simulink model "HRTF_IIR_Baris_FixedPoint_v2"  (R2025a)
settings: Solver=FixedStepDiscrete  StartTime=0.0  StopTime=T_sim  FixedStep=1/48000  RelTol=1e-3
values from neighbouring files (symbols this model uses):
  Alpha = [1 1 0.967796790113 -0.19525471365 0.941178659583 1.27759475775 0.157427422536 -0.232086624749 0.0400536246511 0.488732720219 -0.15013114138 -0.0870474720577 ... (18 elements, 2x9)]    [koeff_parameter_iir.mat]
  Beta = [1 1 4.50665299478 2.25254932437 11.1795102702 3.85997518129 18.0238230447 4.78060301042 20.7495830674 4.97041442912 17.1226318925 4.54493537547 ... (18 elements, 2x9)]    [koeff_parameter_iir.mat]
  Delay = [8966.24819844 7620.20448403]    [koeff_parameter_iir.mat]
  Gain = [4.7297619183 7.71004347236]    [koeff_parameter_iir.mat]
undefined symbols (not defined in the file or in its folder): ALPHA, BETA, DELAY, dspblkCoreblockFVToolHelper, GAIN, gcbh
settings Model: Creator=kucuk  LastModifiedBy=eoencue1
settings OptimizationCC: DefaultParameterBehavior=Inlined  EnhancedBackFolding=on  PassReuseOutputArgsAs=Individual arguments  OptimizeBlockOrder=speed  DifferentSizesBufferReuse=on  OptimizationCustomize=off  EfficientTunableParamExpr=on
settings DebuggingCC: SignalRangeChecking=warning  ParameterTunabilityLossMsg=error
settings HardwareCC: ProdBitPerPointer=32.0  ProdBitPerSizeT=32.0  ProdBitPerPtrDiffT=32.0  ProdLargestAtomicFloat=None  ProdWordSize=32.0  ProdLongLongMode=on  ProdHWDeviceType=Custom Processor->Custom
settings ModelReferenceCC: ModelReferenceNumInstancesAllowed=Single
settings SFSimCC: MATLABDynamicMemAlloc=off
settings RTWCC: SystemTargetFile=ert.tlc  GenCodeOnly=on  TemplateMakefile=ert_default_tmf  Description=Embedded Coder
settings CodeAppCC: ForceParamTrailComments=on  IgnoreCustomStorageClasses=off  OperatorAnnotations=on  SimulinkDataObjDesc=on  SFDataObjDesc=on  InsertBlockDesc=on
settings ERTTargetCC: ExtModeTransport=0.0  ExtModeStaticAlloc=off  ExtModeMexFile=ext_comm  ExtModeIntrfLevel=Level1  ERTCustomFileTemplate=example_file_process.tlc  TargetLangStandard=C99 (ISO)  SubcomponentCodeInterfacePackaging=Nonreusable function  SupportNonFinite=off

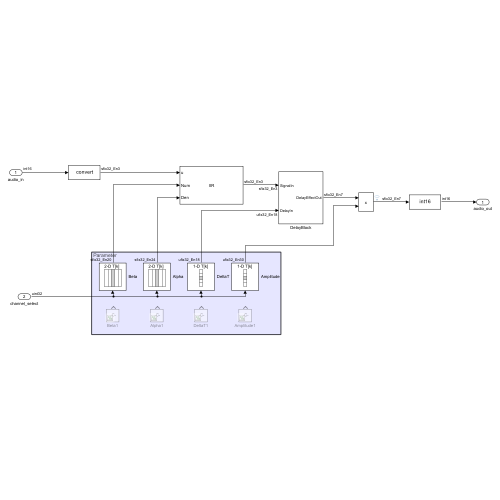
[thumbnail: Simulink's stored preview of the top-level diagram]
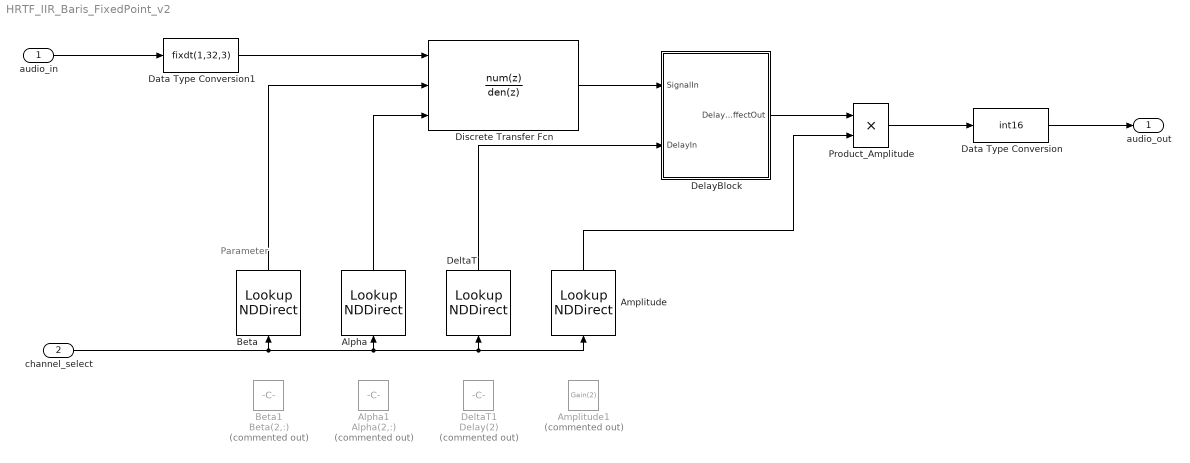
== system HRTF_IIR_Baris_FixedPoint_v2 ==
  note: Parameter
  audio_in : Inport  OutDataTypeStr=int16
  channel_select : Inport  Port=2  OutDataTypeStr=uint32
  Alpha : LookupNDDirect  InputsSelectThisObjectFromTable=Vector  Table=ALPHA  TableDataTypeStr=fixdt(1,32,24)
  Alpha1 : Constant  Commented=on  Value=Alpha(2,:)
  Amplitude : LookupNDDirect  NumberOfTableDimensions=1  Table=GAIN  TableDataTypeStr=fixdt(0,32,30)
  Amplitude1 : Constant  Commented=on  Value=Gain(2)
  Beta : LookupNDDirect  InputsSelectThisObjectFromTable=Vector  Table=BETA  TableDataTypeStr=fixdt(1,32,20)
  Beta1 : Constant  Commented=on  Value=Beta(2,:)
  Data Type Conversion : DataTypeConversion  OutDataTypeStr=int16  RndMeth=Floor
  Data Type Conversion1 : DataTypeConversion  OutDataTypeStr=fixdt(1,32,3)  RndMeth=Floor
  DelayBlock : Subsystem
  DeltaT : LookupNDDirect  NumberOfTableDimensions=1  Table=DELAY  TableDataTypeStr=fixdt(0,32,18)
  DeltaT1 : Constant  Commented=on  Value=Delay(2)
  Discrete Transfer Fcn : DiscreteTransferFcn  LoadFcn=dspblkCoreblockFVToolHelper(gcbh,'load');  NumeratorSource=Input port  DenominatorSource=Input port  a0EqualsOne=on  OutDataTypeStr=fixdt(1,32,3)
      settings: CopyFcn=dspblkCoreblockFVToolHelper(gcbh,'copy');  DeleteFcn=dspblkCoreblockFVToolHelper(gcbh,'close');  ModelCloseFcn=dspblkCoreblockFVToolHelper(gcbh,'close');  PreSaveFcn=dspblkCoreblockFVToolHelper(gcbh,'presave');  PostSaveFcn=dspblkCoreblockFVToolHelper(gcbh,'postsave');  CloseFcn=dspblkCoreblockFVToolHelper(gcbh,'close');  InputPortMap=u0,p1,p3
  Product_Amplitude : Product  OutDataTypeStr=fixdt(1,32,7)
  audio_out : Outport
  wires:
  audio_in/1 -> Data Type Conversion1/1
  Product_Amplitude/1 -> Data Type Conversion/1
  Discrete Transfer Fcn/1 -> DelayBlock/1(SignalIn)
  DelayBlock/1(DelayEffectOut) -> Product_Amplitude/1
  channel_select/1 -> Amplitude/1, DeltaT/1, Alpha/1, Beta/1
  Beta/1 -> Discrete Transfer Fcn/2
  Alpha/1 -> Discrete Transfer Fcn/3
  DeltaT/1 -> DelayBlock/2(DelayIn)
  Amplitude/1 -> Product_Amplitude/2
  Data Type Conversion/1 -> audio_out/1
  Data Type Conversion1/1 -> Discrete Transfer Fcn/1

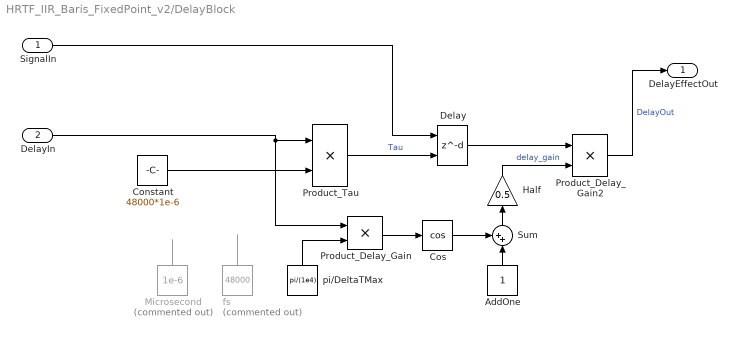
== system HRTF_IIR_Baris_FixedPoint_v2/DelayBlock ==
  SignalIn : Inport  OutDataTypeStr=fixdt(1,32,3)
  DelayIn : Inport  Port=2  OutDataTypeStr=fixdt(0,32,18)
  AddOne : Constant  OutDataTypeStr=fixdt(0,32,31)
  Constant : Constant  Value=48000*1e-6  OutDataTypeStr=fixdt(0,32,36)
  Cos : Trigonometry  Operator=cos  ApproximationMethod=CORDIC
  Delay : Delay  DelayLengthSource=Input port  DelayLengthUpperLimit=10*48000*1e-3  UseCircularBuffer=on
      settings: InputPortMap=u0,p1
  Half : Gain  Gain=0.5  ParamDataTypeStr=fixdt(0,32,32)  OutDataTypeStr=fixdt(0,32,32)
  Microsecond : Constant  Commented=on  Value=1e-6  OutDataTypeStr=fixdt(0,32,51)
  Product_Delay_Gain : Product  OutDataTypeStr=fixdt(0,32,30)
  Product_Delay_Gain2 : Product  OutDataTypeStr=fixdt(1,32,7)
  Product_Tau : Product  OutDataTypeStr=fixdt(0,32,0)
  Sum : Sum  Inputs=++|  OutDataTypeStr=fixdt(0,32,31)  AccumDataTypeStr=fixdt(1,32,30)
  fs : Constant  Commented=on  Value=48000  OutDataTypeStr=fixdt(0,32,16)
  pi/DeltaTMax : Constant  Value=pi/(1e4)  OutDataTypeStr=fixdt(0,32,43)
  DelayEffectOut : Outport
  wires:
  fs/1 -> ?
  Sum/1 -> Half/1
  pi/DeltaTMax/1 -> Product_Delay_Gain/2
  Delay/1 -> Product_Delay_Gain2/1
  Product_Tau/1 -> Delay/2  "Tau"
  Product_Delay_Gain/1 -> Cos/1
  DelayIn/1 -> Product_Delay_Gain/1, Product_Tau/1
  Microsecond/1 -> ?
  AddOne/1 -> Sum/2
  Half/1 -> Product_Delay_Gain2/2  "delay_gain"
  Cos/1 -> Sum/1
  Product_Delay_Gain2/1 -> DelayEffectOut/1  "DelayOut"
  SignalIn/1 -> Delay/1
  Constant/1 -> Product_Tau/2
